simulink model "Assem1"  (R2017a)
settings: Solver=VariableStepAuto  StartTime=0.0  StopTime=10.0  RelTol=1e-3
undefined symbols (not defined in the file or in its folder): base, link1, part1, part2, Part3, part4, Part5
libraries: mblibv1 x18, simulink x4
settings Model: Creator=phoenix  LastModifiedBy=phoenix
settings SimMechanicsCC: VisOnUpdateDiagram=on  VisDuringSimulation=on

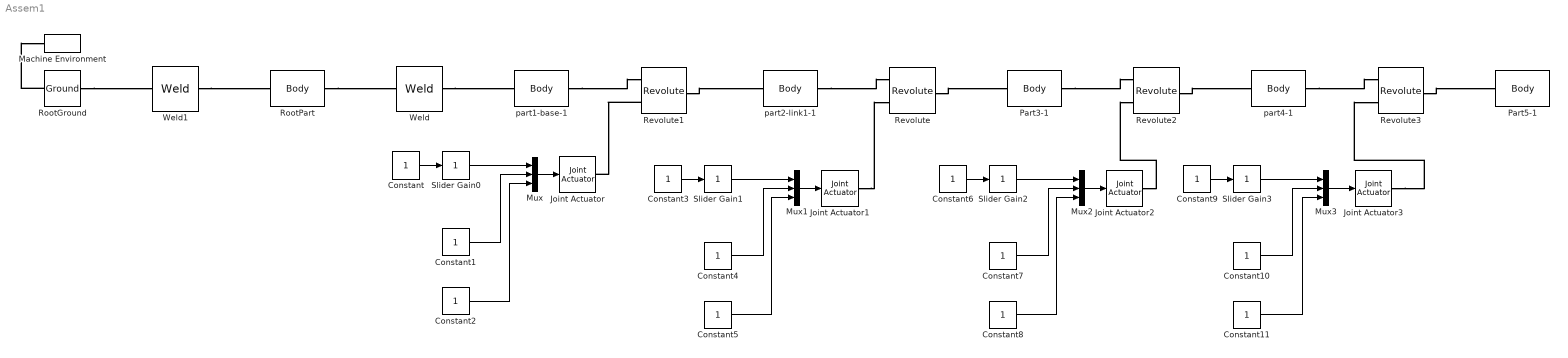
== system Assem1 ==
  Constant{,1..11} (12 alike) : Constant
  Joint Actuator{,1..3} (4 alike) : mblibv1/Sensors &  Actuators/Joint Actuator  UpdateFromCAD=off  PhysicalDomain=Mechanical  PortType=blob  ActuationStyle=Motion  AngleUnits=deg  ArcVelocityUnits=deg/s  ArcAccelerationUnits=deg/s^2  CoordPositionUnits=m  VelocityUnits=m/s  AccelerationUnits=m/s^2  ForceUnits=N  TorqueUnits=N*m  ActiveIO=on  Width=3  DialogClass=MechanicalActuatorBlock  Primitive=R1  ReferenceFrame=Absolute (World)
      settings: SourceProductName=Simscape Multibody  SourceProductBaseCode=MS
  Machine Environment : mblibv1/Bodies/Machine Environment  PortType=env  PhysicalDomain=Mechanical  DialogTemplateClass=MECH.MachineEnvironment  SyncWhenCopied=off  Gravity=[0 -9.81 0]  GravityUnits=m/s^2  GravityAsSignal=off  Dimensionality=Auto-detect  AnalysisType=Forward dynamics  LinearAssemblyTolerance=1e-3  LinearAssemblyToleranceUnits=m  AngularAssemblyTolerance=1e-3  AngularAssemblyToleranceUnits=rad  ConstraintSolverType=Stabilizing  ConstraintRelTolerance=1e-4  ConstraintAbsTolerance=1e-4  UseRobustSingularityHandling=off  RedundancyAnalysisToleranceType=Automatically select tolerance  RedundancyAnalysisTolerance=1e-14  StatePerturbationType=Fixed  PerturbationSize=1e-5  VisualizeMachine=on  BodyVisualizationType=Use model default body geometries  BodyColorSelMode=Use model default  DefaultBodyColor=[1 0 0]
      settings: SourceProductName=Simscape Multibody  SourceProductBaseCode=MS
  Mux{,1..3} (4 alike) : Mux  Inputs=3
  Part3-1 : mblibv1/Bodies/Body  LConnTagsString=CS2  RConnTagsString=CS3  UpdateFromCAD=on  PMImportedID=Part3-1  DialogClass=MechanicalBodyBlock  Mass=15.4829  MassUnits=kg  InertiaUnits=kg*m^2  Inertia=[0.715868,2.21392e-05,-1.41935e-05;2.21392e-05,0.621,0.000259482;-1.41935e-05,0.000259482,0.157371]  Shape=Cylinder  ShapeDims=[1 1]  ShapeUnits=m  ShapeUse=false  Density=1  DensityUnits=kg/m^3  DensityUse=false  GraphicsMode=GFXFILE  GraphicsFileName=Assem1 - Part3-1.STL  BodyColorSelMode=COLORPALETTE  BodyColor=[0.968627;0.878431;0.6]  AttachedToCS=CS1  CG=Right$CG$[0.230857 0.846839 0.447894]$WORLD$WORLD$m$[0.738379 -0.0510776 -0.672448;-0.673327 0 -0.739344;0.0377639 0.998695 -0.0343919]$3x3 Transform$rad$WORLD$false$Part3-1::CG(AUTOGEN)  WorkingFrames=Right$CS1$[0.101976 0.70511 0.441107]$WORLD$WORLD$m$[0.738379 -0.0510776 -0.672448;-0.673327 0 -0.739344;0.0377639 0.998695 -0.0343919]$3x3 Transform$rad$WORLD$false$Part3-1::CS1(AUTOGEN)#Left$CS2$[0.0973794 0.70511 0.530989]$WORLD$WORLD$m$[1 0 0;0 1 0;0 0 1]$3x3 Transform$rad$WORLD$true$Part3-1:-:part2-link1-1::Part3-1(AUTOGEN)#Right$CS3$[0.433604 1.07478 0.548185]$WORLD$WORLD$m$[1 0 0;0 1 0;0 0 1]$3x3 Transform$rad$WORLD$true$Part3-1:-:part4-1::Part3-1(AUTOGEN)  CGPos=[0.230857 0.846839 0.447894]  CGRot=[0.738379 -0.0510776 -0.672448;-0.673327 0 -0.739344;0.0377639 0.998695 -0.0343919]  CS0Pos=[]  CS0Rot=[]  CS1Pos=[0.101976 0.70511 0.441107]  CS1Rot=[0.738379 -0.0510776 -0.672448;-0.673327 0 -0.739344;0.0377639 0.998695 -0.0343919]  CS2Pos=[0.0973794 0.70511 0.530989]  CS2Rot=[1 0 0;0 1 0;0 0 1]  CS3Pos=[0.433604 1.07478 0.548185]  CS3Rot=[1 0 0;0 1 0;0 0 1]  CS4Pos=[]  CS4Rot=[]  CS5Pos=[]  CS5Rot=[]  CS6Pos=[]  CS6Rot=[]  CS7Pos=[]  CS7Rot=[]  CS8Pos=[]  CS8Rot=[]  CS9Pos=[]  CS9Rot=[]  CS10Pos=[]  CS10Rot=[]  CS11Pos=[]  CS11Rot=[]  CS12Pos=[]  CS12Rot=[]  CS13Pos=[]  CS13Rot=[]  CS14Pos=[]  CS14Rot=[]  CS15Pos=[]  CS15Rot=[]  CS16Pos=[]  CS16Rot=[]  CS17Pos=[]  CS17Rot=[]  CS18Pos=[]  CS18Rot=[]  CS19Pos=[]  CS19Rot=[]  CS20Pos=[]  CS20Rot=[]
      settings: SourceProductName=Simscape Multibody  SourceProductBaseCode=MS
  Part5-1 : mblibv1/Bodies/Body  LConnTagsString=CS2  UpdateFromCAD=on  PMImportedID=Part5-1  DialogClass=MechanicalBodyBlock  Mass=1.17548  MassUnits=kg  InertiaUnits=kg*m^2  Inertia=[0.0021374,-1.82283e-09,-4.78629e-11;-1.82283e-09,0.00618923,-1.24661e-09;-4.78629e-11,-1.24661e-09,0.00669914]  Shape=Cylinder  ShapeDims=[1 1]  ShapeUnits=m  ShapeUse=false  Density=1  DensityUnits=kg/m^3  DensityUse=false  GraphicsMode=GFXFILE  GraphicsFileName=Assem1 - Part5-1.STL  BodyColorSelMode=COLORPALETTE  BodyColor=[0.792157;0.819608;0.933333]  AttachedToCS=CS1  CG=Right$CG$[0.833266 1.33043 0.488521]$WORLD$WORLD$m$[0.998466 0.0213822 0.0510776;0.0214101 -0.999771 0;0.0510659 0.00109358 -0.998695]$3x3 Transform$rad$WORLD$false$Part5-1::CG(AUTOGEN)  WorkingFrames=Right$CS1$[0.809555 1.32992 0.487309]$WORLD$WORLD$m$[0.998466 0.0213822 0.0510776;0.0214101 -0.999771 0;0.0510659 0.00109358 -0.998695]$3x3 Transform$rad$WORLD$false$Part5-1::CS1(AUTOGEN)#Left$CS2$[0.807001 1.32992 0.537243]$WORLD$WORLD$m$[1 0 0;0 1 0;0 0 1]$3x3 Transform$rad$WORLD$true$Part5-1:-:part4-1::Part5-1(AUTOGEN)  CGPos=[0.833266 1.33043 0.488521]  CGRot=[0.998466 0.0213822 0.0510776;0.0214101 -0.999771 0;0.0510659 0.00109358 -0.998695]  CS0Pos=[]  CS0Rot=[]  CS1Pos=[0.809555 1.32992 0.487309]  CS1Rot=[0.998466 0.0213822 0.0510776;0.0214101 -0.999771 0;0.0510659 0.00109358 -0.998695]  CS2Pos=[0.807001 1.32992 0.537243]  CS2Rot=[1 0 0;0 1 0;0 0 1]  CS3Pos=[]  CS3Rot=[]  CS4Pos=[]  CS4Rot=[]  CS5Pos=[]  CS5Rot=[]  CS6Pos=[]  CS6Rot=[]  CS7Pos=[]  CS7Rot=[]  CS8Pos=[]  CS8Rot=[]  CS9Pos=[]  CS9Rot=[]  CS10Pos=[]  CS10Rot=[]  CS11Pos=[]  CS11Rot=[]  CS12Pos=[]  CS12Rot=[]  CS13Pos=[]  CS13Rot=[]  CS14Pos=[]  CS14Rot=[]  CS15Pos=[]  CS15Rot=[]  CS16Pos=[]  CS16Rot=[]  CS17Pos=[]  CS17Rot=[]  CS18Pos=[]  CS18Rot=[]  CS19Pos=[]  CS19Rot=[]  CS20Pos=[]  CS20Rot=[]
      settings: SourceProductName=Simscape Multibody  SourceProductBaseCode=MS
  Revolute : mblibv1/Joints/Revolute  LConnTagsString=__newl0|SA1  RConnTagsString=__newr0  UpdateFromCAD=on  PMImportedID=Part3-1:-:part2-link1-1  NumSAPorts=1  CutJoint=off  MarkAsCut=off  Primitives=prismatic  PrimitiveProps=R1$World$[-0.0510776,0,0.998695]$revolute  DialogClass=JointBlock  R1Axis=[-0.0510776,0,0.998695]
      settings: SourceProductName=Simscape Multibody  SourceProductBaseCode=MS
  Revolute1 : mblibv1/Joints/Revolute  LConnTagsString=__newl0|SA1  RConnTagsString=__newr0  UpdateFromCAD=on  PMImportedID=part1-base-1:-:part2-link1-1  NumSAPorts=1  CutJoint=off  MarkAsCut=off  Primitives=prismatic  PrimitiveProps=R1$World$[0,1,0]$revolute  DialogClass=JointBlock  R1Axis=[0,1,0]
      settings: SourceProductName=Simscape Multibody  SourceProductBaseCode=MS
  Revolute2 : mblibv1/Joints/Revolute  LConnTagsString=__newl0|SA1  RConnTagsString=__newr0  UpdateFromCAD=on  PMImportedID=Part3-1:-:part4-1  NumSAPorts=1  CutJoint=off  MarkAsCut=off  Primitives=prismatic  PrimitiveProps=R1$World$[0.0510776,0,-0.998695]$revolute  DialogClass=JointBlock  R1Axis=[0.0510776,0,-0.998695]
      settings: SourceProductName=Simscape Multibody  SourceProductBaseCode=MS
  Revolute3 : mblibv1/Joints/Revolute  LConnTagsString=__newl0|SA1  RConnTagsString=__newr0  UpdateFromCAD=on  PMImportedID=Part5-1:-:part4-1  NumSAPorts=1  CutJoint=off  MarkAsCut=off  Primitives=prismatic  PrimitiveProps=R1$World$[0.0510776,0,-0.998695]$revolute  DialogClass=JointBlock  R1Axis=[0.0510776,0,-0.998695]
      settings: SourceProductName=Simscape Multibody  SourceProductBaseCode=MS
  RootGround : mblibv1/Bodies/Ground  UpdateFromCAD=on  PMImportedID=RootGround  LeftPortType=env  RightPortType=workingframe  PhysicalDomain=Mechanical  DialogClass=GroundBlock  CoordPosition=[0.229995,0.695553,0.459686]  CoordPositionUnits=m  StateVectorMgrId=6  MachineId=[7 0]  ShowEnvPort=on  ParameterChecksum=[3791189980, 16655652, 4278920722, 2420992098]  TopologyChecksum=[1913168167, 4293477489, 1691532797, 981708752]
      settings: SourceProductName=Simscape Multibody  SourceProductBaseCode=MS
  RootPart : mblibv1/Bodies/Body  LConnTagsString=CS3  RConnTagsString=CS2  UpdateFromCAD=on  PMImportedID=Assem1/RootPart  DialogClass=MechanicalBodyBlock  Mass=0  MassUnits=kg  InertiaUnits=kg*m^2  Inertia=[0,0,0;0,0,0;0,0,0]  Shape=Cylinder  ShapeDims=[1 1]  ShapeUnits=m  ShapeUse=false  Density=1  DensityUnits=kg/m^3  DensityUse=false  GraphicsMode=MACHINE_DEFAULT  BodyColorSelMode=MACHINE_DEFAULT  BodyColor=[1;0;0]  AttachedToCS=CS1  CG=Right$CG$[0.229995 0.695553 0.459686]$WORLD$WORLD$m$[1 0 0;0 1 0;0 0 1]$3x3 Transform$rad$WORLD$false$Assem1/RootPart::CG(AUTOGEN)  WorkingFrames=Right$CS1$[0 0 0]$WORLD$WORLD$m$[1 0 0;0 1 0;0 0 1]$3x3 Transform$rad$WORLD$false$Assem1/RootPart::CS1(AUTOGEN)#Right$CS2$[0.101976 0.30232 0.472406]$WORLD$WORLD$m$[1 0 0;0 1 0;0 0 1]$3x3 Transform$rad$WORLD$true$Assem1/RootPart:-:part1-base-1::Assem1/RootPart(AUTOGEN)#Left$CS3$[0.229995 0.695553 0.459686]$WORLD$WORLD$m$[1 0 0;0 1 0;0 0 1]$3x3 Transform$rad$WORLD$true$Assem1/RootPart:-:RootGround::Assem1/RootPart(AUTOGEN)  CGPos=[0.229995 0.695553 0.459686]  CGRot=[1 0 0;0 1 0;0 0 1]  CS0Pos=[]  CS0Rot=[]  CS1Pos=[0 0 0]  CS1Rot=[1 0 0;0 1 0;0 0 1]  CS2Pos=[0.101976 0.30232 0.472406]  CS2Rot=[1 0 0;0 1 0;0 0 1]  CS3Pos=[0.229995 0.695553 0.459686]  CS3Rot=[1 0 0;0 1 0;0 0 1]  CS4Pos=[]  CS4Rot=[]  CS5Pos=[]  CS5Rot=[]  CS6Pos=[]  CS6Rot=[]  CS7Pos=[]  CS7Rot=[]  CS8Pos=[]  CS8Rot=[]  CS9Pos=[]  CS9Rot=[]  CS10Pos=[]  CS10Rot=[]  CS11Pos=[]  CS11Rot=[]  CS12Pos=[]  CS12Rot=[]  CS13Pos=[]  CS13Rot=[]  CS14Pos=[]  CS14Rot=[]  CS15Pos=[]  CS15Rot=[]  CS16Pos=[]  CS16Rot=[]  CS17Pos=[]  CS17Rot=[]  CS18Pos=[]  CS18Rot=[]  CS19Pos=[]  CS19Rot=[]  CS20Pos=[]  CS20Rot=[]
      settings: SourceProductName=Simscape Multibody  SourceProductBaseCode=MS
  Slider Gain{0..3} (4 alike) : simulink/Math Operations/Slider Gain  gain=1  low=-180  high=180
  Weld : mblibv1/Joints/Weld  LConnTagsString=__newl0  RConnTagsString=__newr0  UpdateFromCAD=on  PMImportedID=Assem1/RootPart:-:part1-base-1  NumSAPorts=0  CutJoint=off  MarkAsCut=off  Primitives=weld  PrimitiveProps=W$WORLD$[0.57735,0.57735,0.57735]$weld  DialogClass=JointBlock  WAxis=[0.57735,0.57735,0.57735]
      settings: SourceProductName=Simscape Multibody  SourceProductBaseCode=MS
  Weld1 : mblibv1/Joints/Weld  LConnTagsString=__newl0  RConnTagsString=__newr0  UpdateFromCAD=on  PMImportedID=Assem1/RootPart:-:RootGround  NumSAPorts=0  CutJoint=off  MarkAsCut=off  Primitives=weld  PrimitiveProps=W$WORLD$[0.57735,0.57735,0.57735]$weld  DialogClass=JointBlock  WAxis=[0.57735,0.57735,0.57735]
      settings: SourceProductName=Simscape Multibody  SourceProductBaseCode=MS
  part1-base-1 : mblibv1/Bodies/Body  LConnTagsString=CS2  RConnTagsString=CS3  UpdateFromCAD=on  PMImportedID=part1-base-1  DialogClass=MechanicalBodyBlock  Mass=20.0492  MassUnits=kg  InertiaUnits=kg*m^2  Inertia=[0.424566,6.6415e-08,-2.68762e-08;6.6415e-08,0.498794,-0.0409817;-2.68762e-08,-0.0409817,0.340169]  Shape=Cylinder  ShapeDims=[1 1]  ShapeUnits=m  ShapeUse=false  Density=1  DensityUnits=kg/m^3  DensityUse=false  GraphicsMode=GFXFILE  GraphicsFileName=Assem1 - part1-base-1.STL  BodyColorSelMode=COLORPALETTE  BodyColor=[0.792157;0.819608;0.933333]  AttachedToCS=CS1  CG=Right$CG$[0.101976 0.30232 0.472406]$WORLD$WORLD$m$[1 0 0;0 1 0;0 0 1]$3x3 Transform$rad$WORLD$false$part1-base-1::CG(AUTOGEN)  WorkingFrames=Right$CS1$[0.101976 0.20911 0.441107]$WORLD$WORLD$m$[1 0 0;0 1 0;0 0 1]$3x3 Transform$rad$WORLD$false$part1-base-1::CS1(AUTOGEN)#Left$CS2$[0.101976 0.30232 0.472406]$WORLD$WORLD$m$[1 0 0;0 1 0;0 0 1]$3x3 Transform$rad$WORLD$true$Assem1/RootPart:-:part1-base-1::part1-base-1(AUTOGEN)#Right$CS3$[0.101976 0.48911 0.441107]$WORLD$WORLD$m$[1 0 0;0 1 0;0 0 1]$3x3 Transform$rad$WORLD$true$part1-base-1:-:part2-link1-1::part1-base-1(AUTOGEN)  CGPos=[0.101976 0.30232 0.472406]  CGRot=[1 0 0;0 1 0;0 0 1]  CS0Pos=[]  CS0Rot=[]  CS1Pos=[0.101976 0.20911 0.441107]  CS1Rot=[1 0 0;0 1 0;0 0 1]  CS2Pos=[0.101976 0.30232 0.472406]  CS2Rot=[1 0 0;0 1 0;0 0 1]  CS3Pos=[0.101976 0.48911 0.441107]  CS3Rot=[1 0 0;0 1 0;0 0 1]  CS4Pos=[]  CS4Rot=[]  CS5Pos=[]  CS5Rot=[]  CS6Pos=[]  CS6Rot=[]  CS7Pos=[]  CS7Rot=[]  CS8Pos=[]  CS8Rot=[]  CS9Pos=[]  CS9Rot=[]  CS10Pos=[]  CS10Rot=[]  CS11Pos=[]  CS11Rot=[]  CS12Pos=[]  CS12Rot=[]  CS13Pos=[]  CS13Rot=[]  CS14Pos=[]  CS14Rot=[]  CS15Pos=[]  CS15Rot=[]  CS16Pos=[]  CS16Rot=[]  CS17Pos=[]  CS17Rot=[]  CS18Pos=[]  CS18Rot=[]  CS19Pos=[]  CS19Rot=[]  CS20Pos=[]  CS20Rot=[]
      settings: SourceProductName=Simscape Multibody  SourceProductBaseCode=MS
  part2-link1-1 : mblibv1/Bodies/Body  LConnTagsString=CS3  RConnTagsString=CS2  UpdateFromCAD=on  PMImportedID=part2-link1-1  DialogClass=MechanicalBodyBlock  Mass=14.5147  MassUnits=kg  InertiaUnits=kg*m^2  Inertia=[0.281387,-1.26853e-09,1.25783e-09;-1.26853e-09,0.10949,0;1.25783e-09,0,0.308062]  Shape=Cylinder  ShapeDims=[1 1]  ShapeUnits=m  ShapeUse=false  Density=1  DensityUnits=kg/m^3  DensityUse=false  GraphicsMode=GFXFILE  GraphicsFileName=Assem1 - part2-link1-1.STL  BodyColorSelMode=COLORPALETTE  BodyColor=[0.792157;0.819608;0.933333]  AttachedToCS=CS1  CG=Right$CG$[0.101976 0.582186 0.441107]$WORLD$WORLD$m$[-0.998695 0 0.0510776;0 1 0;-0.0510776 0 -0.998695]$3x3 Transform$rad$WORLD$false$part2-link1-1::CG(AUTOGEN)  WorkingFrames=Right$CS1$[0.101976 0.36911 0.441107]$WORLD$WORLD$m$[-0.998695 0 0.0510776;0 1 0;-0.0510776 0 -0.998695]$3x3 Transform$rad$WORLD$false$part2-link1-1::CS1(AUTOGEN)#Right$CS2$[0.0973794 0.70511 0.530989]$WORLD$WORLD$m$[1 0 0;0 1 0;0 0 1]$3x3 Transform$rad$WORLD$true$Part3-1:-:part2-link1-1::part2-link1-1(AUTOGEN)#Left$CS3$[0.101976 0.48911 0.441107]$WORLD$WORLD$m$[1 0 0;0 1 0;0 0 1]$3x3 Transform$rad$WORLD$true$part1-base-1:-:part2-link1-1::part2-link1-1(AUTOGEN)  CGPos=[0.101976 0.582186 0.441107]  CGRot=[-0.998695 0 0.0510776;0 1 0;-0.0510776 0 -0.998695]  CS0Pos=[]  CS0Rot=[]  CS1Pos=[0.101976 0.36911 0.441107]  CS1Rot=[-0.998695 0 0.0510776;0 1 0;-0.0510776 0 -0.998695]  CS2Pos=[0.0973794 0.70511 0.530989]  CS2Rot=[1 0 0;0 1 0;0 0 1]  CS3Pos=[0.101976 0.48911 0.441107]  CS3Rot=[1 0 0;0 1 0;0 0 1]  CS4Pos=[]  CS4Rot=[]  CS5Pos=[]  CS5Rot=[]  CS6Pos=[]  CS6Rot=[]  CS7Pos=[]  CS7Rot=[]  CS8Pos=[]  CS8Rot=[]  CS9Pos=[]  CS9Rot=[]  CS10Pos=[]  CS10Rot=[]  CS11Pos=[]  CS11Rot=[]  CS12Pos=[]  CS12Rot=[]  CS13Pos=[]  CS13Rot=[]  CS14Pos=[]  CS14Rot=[]  CS15Pos=[]  CS15Rot=[]  CS16Pos=[]  CS16Rot=[]  CS17Pos=[]  CS17Rot=[]  CS18Pos=[]  CS18Rot=[]  CS19Pos=[]  CS19Rot=[]  CS20Pos=[]  CS20Rot=[]
      settings: SourceProductName=Simscape Multibody  SourceProductBaseCode=MS
  part4-1 : mblibv1/Bodies/Body  LConnTagsString=CS2  RConnTagsString=CS3  UpdateFromCAD=on  PMImportedID=part4-1  DialogClass=MechanicalBodyBlock  Mass=12.0871  MassUnits=kg  InertiaUnits=kg*m^2  Inertia=[0.0753981,-0.0400249,0.000341738;-0.0400249,0.339554,4.2814e-05;0.000341738,4.2814e-05,0.371786]  Shape=Cylinder  ShapeDims=[1 1]  ShapeUnits=m  ShapeUse=false  Density=1  DensityUnits=kg/m^3  DensityUse=false  GraphicsMode=GFXFILE  GraphicsFileName=Assem1 - part4-1.STL  BodyColorSelMode=COLORPALETTE  BodyColor=[0.792157;0.819608;0.933333]  AttachedToCS=CS1  CG=Right$CG$[0.536302 1.22843 0.473198]$WORLD$WORLD$m$[0.961521 -0.269943 -0.0510776;0.270296 0.962777 0;0.0491763 -0.0138061 0.998695]$3x3 Transform$rad$WORLD$false$part4-1::CG(AUTOGEN)  WorkingFrames=Right$CS1$[0.309564 1.18937 0.461737]$WORLD$WORLD$m$[0.961521 -0.269943 -0.0510776;0.270296 0.962777 0;0.0491763 -0.0138061 0.998695]$3x3 Transform$rad$WORLD$false$part4-1::CS1(AUTOGEN)#Left$CS2$[0.433604 1.07478 0.548185]$WORLD$WORLD$m$[1 0 0;0 1 0;0 0 1]$3x3 Transform$rad$WORLD$true$Part3-1:-:part4-1::part4-1(AUTOGEN)#Right$CS3$[0.807001 1.32992 0.537243]$WORLD$WORLD$m$[1 0 0;0 1 0;0 0 1]$3x3 Transform$rad$WORLD$true$Part5-1:-:part4-1::part4-1(AUTOGEN)  CGPos=[0.536302 1.22843 0.473198]  CGRot=[0.961521 -0.269943 -0.0510776;0.270296 0.962777 0;0.0491763 -0.0138061 0.998695]  CS0Pos=[]  CS0Rot=[]  CS1Pos=[0.309564 1.18937 0.461737]  CS1Rot=[0.961521 -0.269943 -0.0510776;0.270296 0.962777 0;0.0491763 -0.0138061 0.998695]  CS2Pos=[0.433604 1.07478 0.548185]  CS2Rot=[1 0 0;0 1 0;0 0 1]  CS3Pos=[0.807001 1.32992 0.537243]  CS3Rot=[1 0 0;0 1 0;0 0 1]  CS4Pos=[]  CS4Rot=[]  CS5Pos=[]  CS5Rot=[]  CS6Pos=[]  CS6Rot=[]  CS7Pos=[]  CS7Rot=[]  CS8Pos=[]  CS8Rot=[]  CS9Pos=[]  CS9Rot=[]  CS10Pos=[]  CS10Rot=[]  CS11Pos=[]  CS11Rot=[]  CS12Pos=[]  CS12Rot=[]  CS13Pos=[]  CS13Rot=[]  CS14Pos=[]  CS14Rot=[]  CS15Pos=[]  CS15Rot=[]  CS16Pos=[]  CS16Rot=[]  CS17Pos=[]  CS17Rot=[]  CS18Pos=[]  CS18Rot=[]  CS19Pos=[]  CS19Rot=[]  CS20Pos=[]  CS20Rot=[]
      settings: SourceProductName=Simscape Multibody  SourceProductBaseCode=MS
  wires:
  Constant/1 -> Slider Gain0/1
  Slider Gain0/1 -> Mux/1
  Constant1/1 -> Mux/2
  Constant2/1 -> Mux/3
  Mux/1 -> Joint Actuator/1
  Mux1/1 -> Joint Actuator1/1
  Constant5/1 -> Mux1/3
  Constant4/1 -> Mux1/2
  Slider Gain1/1 -> Mux1/1
  Constant3/1 -> Slider Gain1/1
  Constant6/1 -> Slider Gain2/1
  Slider Gain2/1 -> Mux2/1
  Constant7/1 -> Mux2/2
  Constant8/1 -> Mux2/3
  Mux2/1 -> Joint Actuator2/1
  Mux3/1 -> Joint Actuator3/1
  Constant11/1 -> Mux3/3
  Constant10/1 -> Mux3/2
  Slider Gain3/1 -> Mux3/1
  Constant9/1 -> Slider Gain3/1
  connections:
  RootPart/RConn1 -- Weld/LConn1
  Weld/RConn1 -- part1-base-1/LConn1
  part2-link1-1/RConn1 -- Revolute/LConn1
  Revolute/RConn1 -- Part3-1/LConn1
  part1-base-1/RConn1 -- Revolute1/LConn1
  Revolute1/RConn1 -- part2-link1-1/LConn1
  Part3-1/RConn1 -- Revolute2/LConn1
  Revolute2/RConn1 -- part4-1/LConn1
  part4-1/RConn1 -- Revolute3/LConn1
  Revolute3/RConn1 -- Part5-1/LConn1
  RootGround/RConn1 -- Weld1/LConn1
  Weld1/RConn1 -- RootPart/LConn1
  RootGround/LConn1 -- Machine Environment/RConn1
  Revolute1/LConn2 -- Joint Actuator/RConn1
  Joint Actuator1/RConn1 -- Revolute/LConn2
  Joint Actuator2/RConn1 -- Revolute2/LConn2
  Joint Actuator3/RConn1 -- Revolute3/LConn2
